simulink model "HEMS_1GDL_temperatura"  (R2026b)
settings: Solver=VariableStepAuto  StopTime=5  MaxStep=1e-4
InitFcn:
  | init_HEMS
undefined symbols (not defined in the file): airgap_bp, airgap_zero_current, alpha_cu, beta_Br, beta_ki, C_th, current_bp, d_max, d_min, d_off, Fz_I0, Fz_table, g0, G_cool, I_ff, I_initial, I_max, k_acc, Kd_cur, Kd_pos, Ki_cur, Ki_pos, Kp_cur, Kp_pos, L_coil, m, N_pos, R_coil, T_amb, T_init, t_load, T_ref_mag, T_ref_R, t_step, thermal_on, Ts_cur, Ts_pos, Ts_sens, v_initial, V_max, z_initial
libraries: slpidlib x2
settings Model: Creator=34666  LastModifiedBy=34666

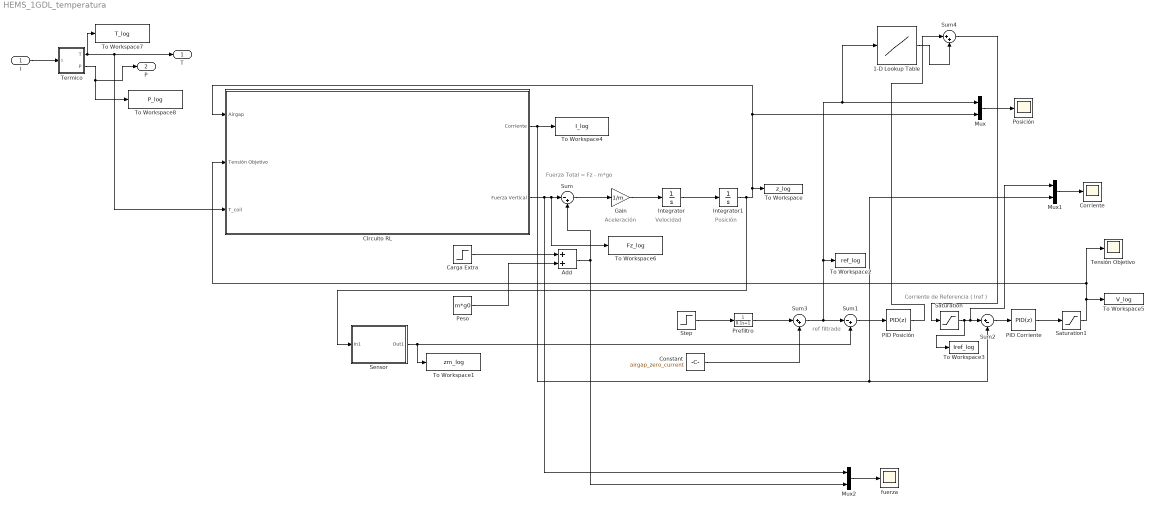
== system HEMS_1GDL_temperatura ==
  note: ref filtrado
  note: Corriente de Referencia ( Iref )
  note: Aceleración
  note: Fuerza Total = Fz - m*go
  note: Velocidad
  note: Posición
  I : Inport
  1-D Lookup Table : Lookup_n-D  NumberOfTableDimensions=1  BreakpointsForDimension1=airgap_bp  Table=I_ff  ExtrapMethod=Clip  InternalRulePriority=Speed  RndMeth=Simplest
  Add : Sum
  CIrcuito RL : Subsystem
  "Carga Extra " : Step  Time=t_load  FinalValue=F_load  SampleTime=0
  Constant : Constant  Value=airgap_zero_current
  Corriente : Scope
      settings: ActiveDisplayYMinimum=-10.906431970254681  ActiveDisplayYMaximum=11.23806537043046  DataLoggingVariableName=ScopeData2
  Gain : Gain  Gain=1/m
  Integrator : Integrator  InitialCondition=v_initial
  Integrator1 : Integrator  InitialCondition=z_initial
  Mux : Mux  Inputs=2
  Mux1 : Mux  Inputs=2
  Mux2 : Mux  Inputs=2
  PID Corriente : slpidlib/PID Controller  Controller=PID  Form=Parallel  TimeDomain=Discrete-time  UseExternalTs=off  SampleTime=Ts_cur  IntegratorMethod=Forward Euler  FilterMethod=Forward Euler  ControllerParametersSource=internal  P=Kp_cur  I=Ki_cur  UseKiTs=off  D=Kd_cur  UseExternalDerivativeSource=off  N=100  UseFilter=on  TunerSelectOption=Transfer Function Based (PID Tuner App)  InitialConditionSource=internal  InitialConditionForIntegrator=0  InitialConditionForFilter=0  DifferentiatorICPrevScaledInput=0  ExternalReset=none  TrackingMode=off  Kt=1  LimitOutput=on  SatLimitsSource=internal  UpperSaturationLimit=V_max  LowerSaturationLimit=-V_max  LinearizeAsGain=on  AntiWindupMode=back-calculation  Kb=1  LimitIntegrator=off  UpperIntegratorSaturationLimit=inf  LowerIntegratorSaturationLimit=-inf  POutMin=[]  POutMax=[]  IOutMin=[]  IOutMax=[]  DOutMin=[]  DOutMax=[]  NOutMin=[]  NOutMax=[]  SumOutMin=[]  SumOutMax=[]  SaturationOutMin=[]  SaturationOutMax=[]  PParamMin=[]  PParamMax=[]  IParamMin=[]  IParamMax=[]  DParamMin=[]  DParamMax=[]  NParamMin=[]  NParamMax=[]  KbParamMin=[]  KbParamMax=[]  KtParamMin=[]  KtParamMax=[]  KbOutMin=[]  KbOutMax=[]  KtOutMin=[]  KtOutMax=[]  IntegratorOutMin=[]  IntegratorOutMax=[]  FilterOutMin=[]  FilterOutMax=[]  SumI1OutMin=[]  SumI1OutMax=[]  SumI2OutMin=[]  SumI2OutMax=[]  SumI3OutMin=[]  SumI3OutMax=[]  SumI4OutMin=[]  SumI4OutMax=[]  SumDOutMin=[]  SumDOutMax=[]  DifferentiatorOutMin=[]  DifferentiatorOutMax=[]  FilterDiffOutCoefMin=[]  FilterDiffOutCoefMax=[]  ReciprocalOutMin=[]  ReciprocalOutMax=[]  SumDenOutMin=[]  SumDenOutMax=[]  SumNumOutMin=[]  SumNumOutMax=[]  DivideOutMin=[]  DivideOutMax=[]  UdiffTsProdOutMin=[]  UdiffTsProdOutMax=[]  NTsProdOutMin=[]  NTsProdOutMax=[]  UintegralTsProdOutMin=[]  UintegralTsProdOutMax=[]  UngainTsProdOutMin=[]  UngainTsProdOutMax=[]  ClampingZeroOutDataTypeStr=Inherit: Inherit via back propagation  ClampingZeroOutMin=[]  ClampingZeroOutMax=[]  FilterDenConstantOutDataTypeStr=Inherit: Inherit via back propagation  FilterDenConstantOutMin=[]  FilterDenConstantOutMax=[]  PCopyOutDataTypeStr=Inherit: Inherit via back propagation  PCopyOutMin=[]  PCopyOutMax=[]  NCopyOutDataTypeStr=Inherit: Inherit via back propagation  NCopyOutMin=[]  NCopyOutMax=[]  IntegratorContinuousStateAttributes=''  IntegratorStateMustResolveToSignalObject=off  IntegratorRTWStateStorageClass=Auto  FilterContinuousStateAttributes=''  FilterStateMustResolveToSignalObject=off  FilterRTWStateStorageClass=Auto  ParallelPVariant=InternalParameters  IdealPVariant=Disabled  IVariant=InternalParameters  DVariant=InternalParameters  IntegratorVariant=Discrete  SatVariant=Enabled  AWVariant=BackCalculation  PCopyVariant=Disabled  TRVariant=Disabled  FdbkBlocksVariant=Forward  IdealPFdbkVariant=Disabled  SatFdbkVariant=Disabled  DerivativeFilterVariant=ForwardEulerFilter  NVariant=InternalParameters  NCopyVariant=Disabled  FilterICVariant=InternalICsFilter  IntegratorICVariant=InternalICs  ExternalResetVariant=Disabled  TRSumVariant=Passthrough  SumFdbkVariant=Disabled  SumVariant=Sum_PID  TsampFilterVariant=InternalTs  TsampNgainVariant=Passthrough  TsampIntegralVariant=Disabled_SignalSpec  ExternalSaturationOutDataTypeStr=Inherit: Same as second input  DerivativeSourceVariant=ErrorSignal  PreIntVariant=InternalPreInt
  PID Posición : slpidlib/PID Controller  Controller=PID  Form=Parallel  TimeDomain=Discrete-time  UseExternalTs=off  SampleTime=Ts_pos  IntegratorMethod=Forward Euler  FilterMethod=Forward Euler  ControllerParametersSource=internal  P=Kp_pos  I=Ki_pos  UseKiTs=off  D=Kd_pos  UseExternalDerivativeSource=off  N=N_pos  UseFilter=on  TunerSelectOption=Transfer Function Based (PID Tuner App)  InitialConditionSource=internal  InitialConditionForIntegrator=0  InitialConditionForFilter=0  DifferentiatorICPrevScaledInput=0  ExternalReset=none  TrackingMode=off  Kt=1  LimitOutput=on  SatLimitsSource=internal  UpperSaturationLimit=I_max  LowerSaturationLimit=-I_max  LinearizeAsGain=on  AntiWindupMode=back-calculation  Kb=1  LimitIntegrator=off  UpperIntegratorSaturationLimit=inf  LowerIntegratorSaturationLimit=-inf  POutMin=[]  POutMax=[]  IOutMin=[]  IOutMax=[]  DOutMin=[]  DOutMax=[]  NOutMin=[]  NOutMax=[]  SumOutMin=[]  SumOutMax=[]  SaturationOutMin=[]  SaturationOutMax=[]  PParamMin=[]  PParamMax=[]  IParamMin=[]  IParamMax=[]  DParamMin=[]  DParamMax=[]  NParamMin=[]  NParamMax=[]  KbParamMin=[]  KbParamMax=[]  KtParamMin=[]  KtParamMax=[]  KbOutMin=[]  KbOutMax=[]  KtOutMin=[]  KtOutMax=[]  IntegratorOutMin=[]  IntegratorOutMax=[]  FilterOutMin=[]  FilterOutMax=[]  SumI1OutMin=[]  SumI1OutMax=[]  SumI2OutMin=[]  SumI2OutMax=[]  SumI3OutMin=[]  SumI3OutMax=[]  SumI4OutMin=[]  SumI4OutMax=[]  SumDOutMin=[]  SumDOutMax=[]  DifferentiatorOutMin=[]  DifferentiatorOutMax=[]  FilterDiffOutCoefMin=[]  FilterDiffOutCoefMax=[]  ReciprocalOutMin=[]  ReciprocalOutMax=[]  SumDenOutMin=[]  SumDenOutMax=[]  SumNumOutMin=[]  SumNumOutMax=[]  DivideOutMin=[]  DivideOutMax=[]  UdiffTsProdOutMin=[]  UdiffTsProdOutMax=[]  NTsProdOutMin=[]  NTsProdOutMax=[]  UintegralTsProdOutMin=[]  UintegralTsProdOutMax=[]  UngainTsProdOutMin=[]  UngainTsProdOutMax=[]  ClampingZeroOutDataTypeStr=Inherit: Inherit via back propagation  ClampingZeroOutMin=[]  ClampingZeroOutMax=[]  FilterDenConstantOutDataTypeStr=Inherit: Inherit via back propagation  FilterDenConstantOutMin=[]  FilterDenConstantOutMax=[]  PCopyOutDataTypeStr=Inherit: Inherit via back propagation  PCopyOutMin=[]  PCopyOutMax=[]  NCopyOutDataTypeStr=Inherit: Inherit via back propagation  NCopyOutMin=[]  NCopyOutMax=[]  IntegratorContinuousStateAttributes=''  IntegratorStateMustResolveToSignalObject=off  IntegratorRTWStateStorageClass=Auto  FilterContinuousStateAttributes=''  FilterStateMustResolveToSignalObject=off  FilterRTWStateStorageClass=Auto  ParallelPVariant=InternalParameters  IdealPVariant=Disabled  IVariant=InternalParameters  DVariant=InternalParameters  IntegratorVariant=Discrete  SatVariant=Enabled  AWVariant=BackCalculation  PCopyVariant=Disabled  TRVariant=Disabled  FdbkBlocksVariant=Forward  IdealPFdbkVariant=Disabled  SatFdbkVariant=Disabled  DerivativeFilterVariant=ForwardEulerFilter  NVariant=InternalParameters  NCopyVariant=Disabled  FilterICVariant=InternalICsFilter  IntegratorICVariant=InternalICs  ExternalResetVariant=Disabled  TRSumVariant=Passthrough  SumFdbkVariant=Disabled  SumVariant=Sum_PID  TsampFilterVariant=InternalTs  TsampNgainVariant=Passthrough  TsampIntegralVariant=Disabled_SignalSpec  ExternalSaturationOutDataTypeStr=Inherit: Same as second input  DerivativeSourceVariant=ErrorSignal  PreIntVariant=InternalPreInt
  Peso : Constant  Value=m*g0
  Posición : Scope
      settings: ActiveDisplayYMinimum=0.01627428772982192  ActiveDisplayYMaximum=0.018331043916801626
  Prefiltro : TransferFcn  Denominator=[0.1 1]
  Saturation : Saturate  UpperLimit=I_max  LowerLimit=-I_max
  Saturation1 : Saturate  UpperLimit=V_max  LowerLimit=-V_max
  Sensor : Subsystem
  Step : Step  Time=t_step  FinalValue=0.018-airgap_zero_current  SampleTime=0
  Sum : Sum  Inputs=|-+
  Sum1 : Sum  Inputs=|-+
  Sum2 : Sum  Inputs=|+-
  Sum3 : Sum  Inputs=|++
  Sum4 : Sum  Inputs=|++
  Tensión Objetivo : Scope
      settings: ActiveDisplayYMinimum=-9.5817260475017871  ActiveDisplayYMaximum=18.365783425274739
  Termico : Subsystem
  To Workspace : ToWorkspace  VariableName=z_log  SaveFormat=Timeseries  SampleTime=-1
  To Workspace1 : ToWorkspace  VariableName=zm_log  SaveFormat=Timeseries  SampleTime=-1
  To Workspace2 : ToWorkspace  VariableName=ref_log  SaveFormat=Timeseries  SampleTime=-1
  To Workspace3 : ToWorkspace  VariableName=Iref_log  SaveFormat=Timeseries  SampleTime=-1
  To Workspace4 : ToWorkspace  VariableName=I_log  SaveFormat=Timeseries  SampleTime=-1
  To Workspace5 : ToWorkspace  VariableName=V_log  SaveFormat=Timeseries  SampleTime=-1
  To Workspace6 : ToWorkspace  VariableName=Fz_log  SaveFormat=Timeseries  SampleTime=-1
  To Workspace7 : ToWorkspace  VariableName=T_log  SaveFormat=Timeseries  SampleTime=-1
  To Workspace8 : ToWorkspace  VariableName=P_log  SaveFormat=Timeseries  SampleTime=-1
  fuerza : Scope
      settings: ActiveDisplayYMinimum=349.8545191819162  ActiveDisplayYMaximum=731.51535099662465  DataLoggingVariableName=ScopeData3
  T : Outport
  P : Outport  Port=2
  wires:
  CIrcuito RL/2(Fuerza Vertical) -> Mux2/1, To Workspace6/1, Sum/1
  Sum/1 -> Gain/1
  Gain/1 -> Integrator/1
  Integrator/1 -> Integrator1/1
  Integrator1/1 -> Sensor/1(In1), Mux/2, CIrcuito RL/1(Airgap), To Workspace/1
  Sum1/1 -> PID Posición/1
  Saturation/1 -> To Workspace3/1, Mux1/1, Sum2/1
  CIrcuito RL/1("Corriente ") -> To Workspace4/1, Sum2/2, Mux1/2
  Sum2/1 -> PID Corriente/1
  PID Corriente/1 -> Saturation1/1
  Saturation1/1 -> Tensión Objetivo/1, CIrcuito RL/2("Tensión Objetivo "), To Workspace5/1
  Mux/1 -> Posición/1
  Mux1/1 -> Corriente/1
  Mux2/1 -> fuerza/1
  Step/1 -> Prefiltro/1
  Prefiltro/1 -> Sum3/1
  Constant/1 -> Sum3/2
  Sum3/1 -> 1-D Lookup Table/1, Mux/1, To Workspace2/1, Sum1/1
  PID Posición/1 -> Sum4/1
  1-D Lookup Table/1 -> Sum4/2
  Sum4/1 -> Saturation/1
  Sensor/1(Out1) -> To Workspace1/1, Sum1/2
  I/1 -> Termico/1(I)
  Termico/1(T) -> CIrcuito RL/3(T_coil), T/1, To Workspace7/1
  Termico/2(P) -> To Workspace8/1, P/1
  "Carga Extra "/1 -> Add/1
  Peso/1 -> Add/2
  Add/1 -> Mux2/2, Sum/2

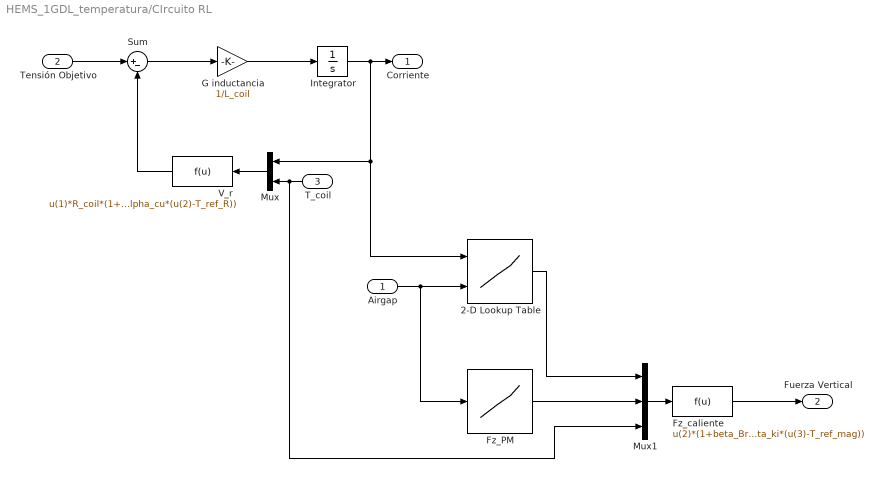
== system HEMS_1GDL_temperatura/CIrcuito RL ==
  Airgap : Inport
  "Tensión Objetivo " : Inport  Port=2
  T_coil : Inport  Port=3
  2-D Lookup Table : Lookup_n-D  BreakpointsForDimension1=current_bp  BreakpointsForDimension2=airgap_bp  Table=Fz_table  ExtrapMethod=Clip  InternalRulePriority=Speed  RndMeth=Simplest
      settings: InputPortMap=u0,u1
  Fz_PM : Lookup_n-D  NumberOfTableDimensions=1  BreakpointsForDimension1=airgap_bp  Table=Fz_I0  ExtrapMethod=Clip  InternalRulePriority=Speed  RndMeth=Simplest
  Fz_caliente : Fcn  Expr=u(2)*(1+beta_Br*(u(3)-T_ref_mag)) + (u(1)-u(2))*(1+beta_ki*(u(3)-T_ref_mag))
  G inductancia : Gain  Gain=1/L_coil
  Integrator : Integrator  InitialCondition=I_initial
  Mux : Mux  Inputs=2
  Mux1 : Mux  Inputs=3
  Sum : Sum  Inputs=|+-
  V_r : Fcn  Expr=u(1)*R_coil*(1+alpha_cu*(u(2)-T_ref_R))
  "Corriente " : Outport
  Fuerza Vertical : Outport  Port=2
  wires:
  "Tensión Objetivo "/1 -> Sum/1
  Sum/1 -> G inductancia/1
  G inductancia/1 -> Integrator/1
  Integrator/1 -> Mux/1, 2-D Lookup Table/1, "Corriente "/1
  Airgap/1 -> Fz_PM/1, 2-D Lookup Table/2
  2-D Lookup Table/1 -> Mux1/1
  T_coil/1 -> Mux1/3, Mux/2
  Mux/1 -> V_r/1
  V_r/1 -> Sum/2
  Fz_PM/1 -> Mux1/2
  Mux1/1 -> Fz_caliente/1
  Fz_caliente/1 -> Fuerza Vertical/1

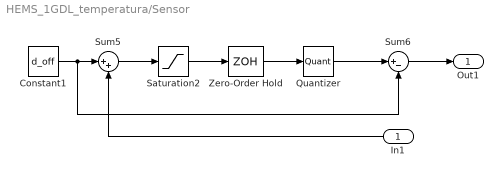
== system HEMS_1GDL_temperatura/Sensor ==
  In1 : Inport
  Constant1 : Constant  Value=d_off
  Quantizer : Quantizer  QuantizationInterval=q_sens
  Saturation2 : Saturate  UpperLimit=d_max  LowerLimit=d_min
  Sum5 : Sum  Inputs=|++
  Sum6 : Sum  Inputs=|+-
  Zero-Order Hold : ZeroOrderHold  SampleTime=Ts_sens
  Out1 : Outport
  wires:
  Quantizer/1 -> Sum6/1
  In1/1 -> Sum5/2
  Sum5/1 -> Saturation2/1
  Constant1/1 -> Sum5/1, Sum6/2
  Saturation2/1 -> Zero-Order Hold/1
  Zero-Order Hold/1 -> Quantizer/1
  Sum6/1 -> Out1/1

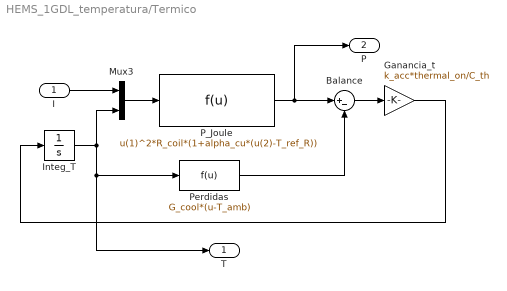
== system HEMS_1GDL_temperatura/Termico ==
  I : Inport
  Balance : Sum  Inputs=|+-
  Ganancia_t : Gain  Gain=k_acc*thermal_on/C_th
  Integ_T : Integrator  InitialCondition=T_init
  Mux3 : Mux  Inputs=2
  P_Joule : Fcn  Expr=u(1)^2*R_coil*(1+alpha_cu*(u(2)-T_ref_R))
  Perdidas : Fcn  Expr=G_cool*(u-T_amb)
  T : Outport
  P : Outport  Port=2
  wires:
  I/1 -> Mux3/1
  Integ_T/1 -> T/1, Perdidas/1, Mux3/2
  Perdidas/1 -> Balance/2
  Mux3/1 -> P_Joule/1
  Ganancia_t/1 -> Integ_T/1
  P_Joule/1 -> P/1, Balance/1
  Balance/1 -> Ganancia_t/1
